simulink model "kalman_beginner_2d"  (R2025b)
settings: Solver=FixedStepDiscrete  StartTime=0.0  StopTime=30  FixedStep=0.1  RelTol=1e-3
model workspace (MAT data in the model file):
  A = [1  0.1; 0  1]
  H = [1 0]
  Q = [0.001  0; 0  0.0001]
  R = 0.25
settings Model: Creator=alosw  LastModifiedBy=alosw

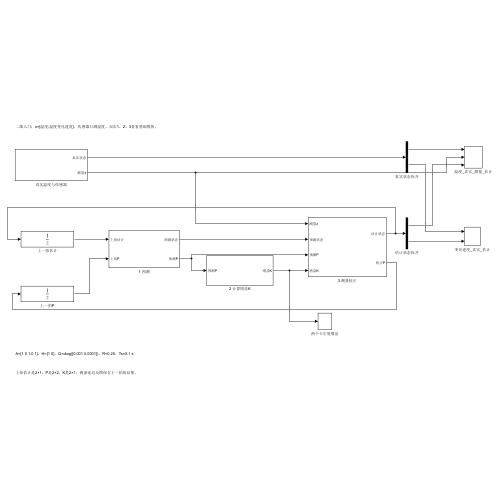
[thumbnail: Simulink's stored preview of the top-level diagram]
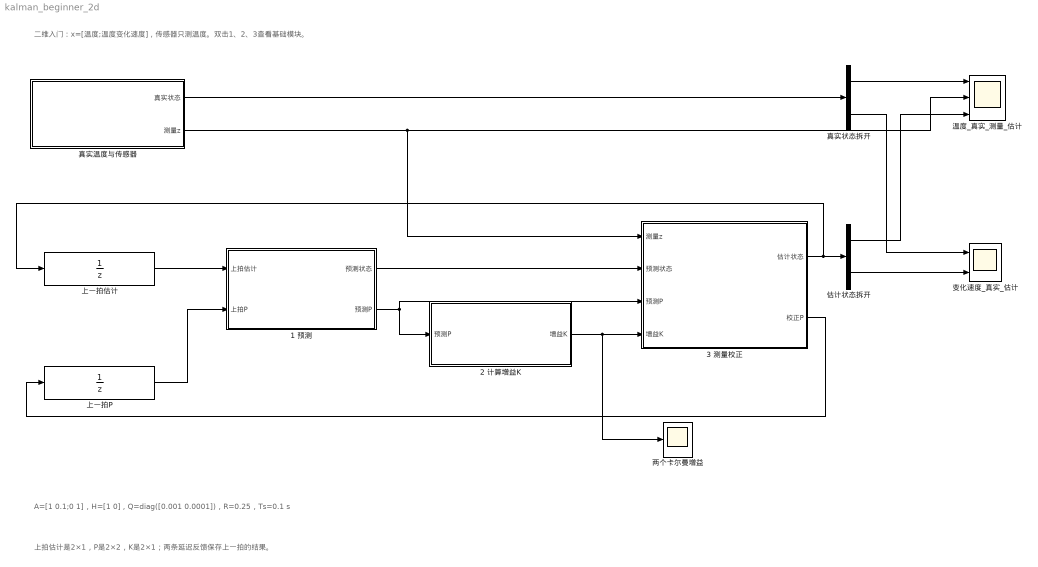
== system kalman_beginner_2d ==
  note: 二维入门：x=[温度;温度变化速度]，传感器只测温度。双击1、2、3查看基础模块。
  note: A=[1 0.1;0 1]，H=[1 0]，Q=diag([0.001 0.0001])，R=0.25，Ts=0.1 s
  note: 上拍估计是2×1，P是2×2，K是2×1；两条延迟反馈保存上一拍的结果。
  1 预测 : Subsystem
  2 计算增益K : Subsystem
  3 测量校正 : Subsystem
  上一拍P : UnitDelay  InitialCondition=diag([4 1])  SampleTime=0.1  HasFrameUpgradeWarning=on
  上一拍估计 : UnitDelay  InitialCondition=[18;0]  SampleTime=0.1  HasFrameUpgradeWarning=on
  两个卡尔曼增益 : Scope
  估计状态拆开 : Demux  Outputs=2
  变化速度_真实_估计 : Scope  NumInputPorts=2
  温度_真实_测量_估计 : Scope  NumInputPorts=3
  真实温度与传感器 : Subsystem
  真实状态拆开 : Demux  Outputs=2
  wires:
  真实温度与传感器/1(真实状态) -> 真实状态拆开/1
  真实温度与传感器/2(测量z) -> 3 测量校正/1(测量z), 温度_真实_测量_估计/2
  上一拍估计/1 -> 1 预测/1(上拍估计)
  上一拍P/1 -> 1 预测/2(上拍P)
  1 预测/1(预测状态) -> 3 测量校正/2(预测状态)
  1 预测/2(预测P) -> 3 测量校正/3(预测P), 2 计算增益K/1(预测P)
  2 计算增益K/1(增益K) -> 两个卡尔曼增益/1, 3 测量校正/4(增益K)
  3 测量校正/1(估计状态) -> 估计状态拆开/1, 上一拍估计/1
  3 测量校正/2(校正P) -> 上一拍P/1
  真实状态拆开/1 -> 温度_真实_测量_估计/1
  估计状态拆开/1 -> 温度_真实_测量_估计/3
  真实状态拆开/2 -> 变化速度_真实_估计/1
  估计状态拆开/2 -> 变化速度_真实_估计/2

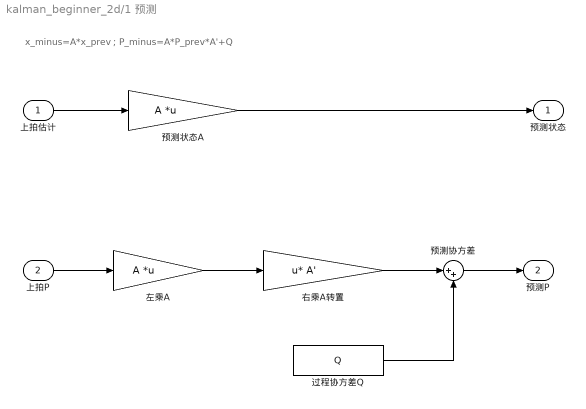
== system kalman_beginner_2d/1 预测 ==
  note: x_minus=A*x_prev；P_minus=A*P_prev*A'+Q
  上拍估计 : Inport
  上拍P : Inport  Port=2
  右乘A转置 : Gain  Gain=A'  Multiplication=Matrix(u*K)
  左乘A : Gain  Gain=A  Multiplication=Matrix(K*u)
  过程协方差Q : Constant  Value=Q
  预测协方差 : Sum  Inputs=|++
  预测状态A : Gain  Gain=A  Multiplication=Matrix(K*u)
  预测状态 : Outport
  预测P : Outport  Port=2
  wires:
  上拍估计/1 -> 预测状态A/1
  预测状态A/1 -> 预测状态/1
  上拍P/1 -> 左乘A/1
  左乘A/1 -> 右乘A转置/1
  右乘A转置/1 -> 预测协方差/1
  过程协方差Q/1 -> 预测协方差/2
  预测协方差/1 -> 预测P/1

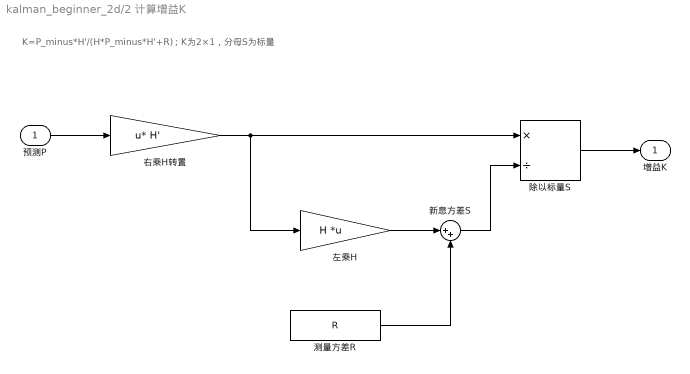
== system kalman_beginner_2d/2 计算增益K ==
  note: K=P_minus*H'/(H*P_minus*H'+R)；K为2×1，分母S为标量
  预测P : Inport
  右乘H转置 : Gain  Gain=H'  Multiplication=Matrix(u*K)
  左乘H : Gain  Gain=H  Multiplication=Matrix(K*u)
  新息方差S : Sum  Inputs=|++
  测量方差R : Constant  Value=R
  除以标量S : Product  Inputs=*/
  增益K : Outport
  wires:
  预测P/1 -> 右乘H转置/1
  右乘H转置/1 -> 除以标量S/1, 左乘H/1
  左乘H/1 -> 新息方差S/1
  测量方差R/1 -> 新息方差S/2
  新息方差S/1 -> 除以标量S/2
  除以标量S/1 -> 增益K/1

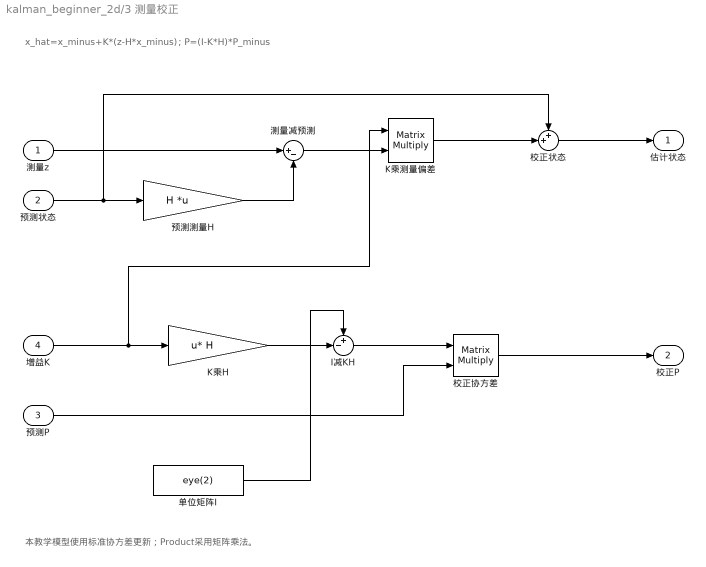
== system kalman_beginner_2d/3 测量校正 ==
  note: x_hat=x_minus+K*(z-H*x_minus)；P=(I-K*H)*P_minus
  note: 本教学模型使用标准协方差更新；Product采用矩阵乘法。
  测量z : Inport
  预测状态 : Inport  Port=2
  预测P : Inport  Port=3
  增益K : Inport  Port=4
  I减KH : Sum  Inputs=+-|
  K乘H : Gain  Gain=H  Multiplication=Matrix(u*K)
  K乘测量偏差 : Product  Inputs=**  Multiplication=Matrix(*)
  单位矩阵I : Constant  Value=eye(2)
  校正协方差 : Product  Inputs=**  Multiplication=Matrix(*)
  校正状态 : Sum  Inputs=++|
  测量减预测 : Sum  Inputs=|+-
  预测测量H : Gain  Gain=H  Multiplication=Matrix(K*u)
  估计状态 : Outport
  校正P : Outport  Port=2
  wires:
  测量z/1 -> 测量减预测/1
  预测状态/1 -> 预测测量H/1, 校正状态/1
  预测测量H/1 -> 测量减预测/2
  增益K/1 -> K乘测量偏差/1, K乘H/1
  测量减预测/1 -> K乘测量偏差/2
  K乘测量偏差/1 -> 校正状态/2
  校正状态/1 -> 估计状态/1
  单位矩阵I/1 -> I减KH/1
  K乘H/1 -> I减KH/2
  I减KH/1 -> 校正协方差/1
  预测P/1 -> 校正协方差/2
  校正协方差/1 -> 校正P/1

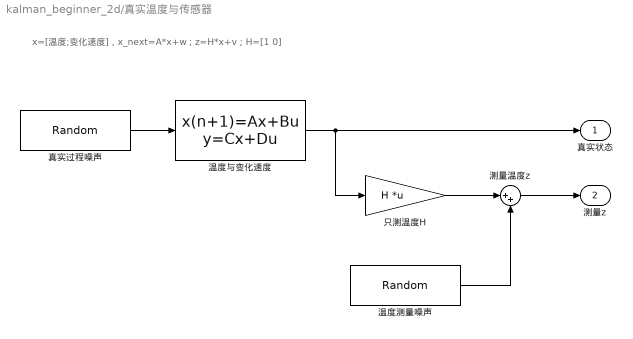
== system kalman_beginner_2d/真实温度与传感器 ==
  note: x=[温度;变化速度]，x_next=A*x+w；z=H*x+v；H=[1 0]
  只测温度H : Gain  Gain=H  Multiplication=Matrix(K*u)
  测量温度z : Sum  Inputs=|++
  温度与变化速度 : DiscreteStateSpace  A=A  B=eye(2)  C=eye(2)  D=zeros(2)  InitialCondition=[20;0.1]  SampleTime=0.1
  温度测量噪声 : RandomNumber  Variance=R  Seed=5678  SampleTime=0.1
  真实过程噪声 : RandomNumber  Mean=[0;0]  Variance=[0.001;0.0001]  Seed=[1234;4321]  SampleTime=0.1
  真实状态 : Outport
  测量z : Outport  Port=2
  wires:
  真实过程噪声/1 -> 温度与变化速度/1
  温度与变化速度/1 -> 真实状态/1, 只测温度H/1
  只测温度H/1 -> 测量温度z/1
  温度测量噪声/1 -> 测量温度z/2
  测量温度z/1 -> 测量z/1
